simulink model "Kirov_physics"  (R2024b)
settings: Solver=FixedStepDiscrete  StartTime=0.0  StopTime=inf  FixedStep=dt  RelTol=1e-3
undefined symbols (not defined in the file): accel_O, airspeed_bp, alpha_B, alpha_bp, alphaFull, alphaOff, b, battery_capacity_bp, battery_current_bp, battery_initial_capacity_mAh, battery_voltage_table, beta_bp, betaFull, betaOff, brake, brakes, c, channels, CLa, Clb, Clp, CLq, Clr, Cma, Cmq, Cnb, Cnp, Cnr, current_table, DiscIntNeverNeededParam, dt, ELEV_bp, elevator, f, flap, flaps, FLAPS_bp, gear, heightFadeStart, heightOff, hgt_0, Inertia_body, Inertia_load, kInduced, L_aileron, L_throttle, LAILE_bp, lat_0, lon_0, M_aile, M_body, M_elev, M_flap, M_front_gear, M_load, M_main_gear, M_prop, M_rudd, M_spoiler, minWingHeight ... (+36)
libraries: sm_lib x673, simulink x58, nesl_utility x51, simulink_extras x24, uavmavlinklib x12, instrumentlib x4, vrlib x3, aerolibfltsims x3, sharedtransform x3, eeGeneralControl x2, aerolibutil x2, AP_Connector x2
(part 6 of 6)

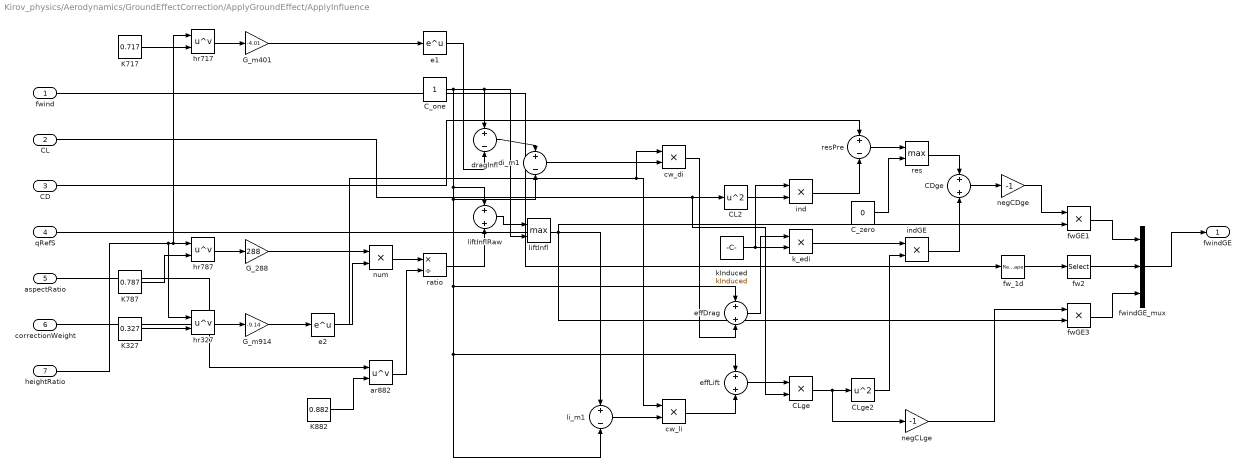
== system Kirov_physics/Aerodynamics/GroundEffectCorrection/ApplyGroundEffect/ApplyInfluence ==
  fwind : Inport
  CL : Inport  Port=2
  CD : Inport  Port=3
  qRefS : Inport  Port=4
  aspectRatio : Inport  Port=5
  correctionWeight : Inport  Port=6
  heightRatio : Inport  Port=7
  CDge : Sum
  CL2 : Math  Operator=square
  CLge : Product
  CLge2 : Math  Operator=square
  C_one : Constant
  C_zero : Constant  Value=0
  G_288 : Gain  Gain=288
  G_m401 : Gain  Gain=-4.01
  G_m914 : Gain  Gain=-9.14
  K327 : Constant  Value=0.327
  K717 : Constant  Value=0.717
  K787 : Constant  Value=0.787
  K882 : Constant  Value=0.882
  ar882 : Math  Operator=pow
  cw_di : Product
  cw_li : Product
  di_m1 : Sum  Inputs=+-
  dragInfl : Sum  Inputs=+-
  e1 : Math
  e2 : Math
  effDrag : Sum
  effLift : Sum
  fw2 : Selector  InputPortWidth=3  IndexOptions=Index vector (dialog)  Indices=[2]  OutputSizes=1
  fwGE1 : Product
  fwGE3 : Product
  fw_1d : Reshape
  fwindGE_mux : Mux  Inputs=3
  hr327 : Math  Operator=pow
  hr717 : Math  Operator=pow
  hr787 : Math  Operator=pow
  ind : Product
  indGE : Product
  kInduced : Constant  Value=kInduced
  k_edi : Product
  li_m1 : Sum  Inputs=+-
  liftInfl : MinMax  Function=max  Inputs=2
  liftInflRaw : Sum
  negCDge : Gain  Gain=-1
  negCLge : Gain  Gain=-1
  num : Product
  ratio : Product  Inputs=*/
  res : MinMax  Function=max  Inputs=2
  resPre : Sum  Inputs=+-
  fwindGE : Outport
  wires:
  hr717/1 -> G_m401/1
  fwGE3/1 -> fwindGE_mux/3
  CL2/1 -> ind/2
  heightRatio/1 -> hr327/1, hr717/1, hr787/1
  C_one/1 -> effLift/1, li_m1/2, effDrag/1, di_m1/2, liftInflRaw/1, liftInfl/2, dragInfl/1
  K717/1 -> hr717/2
  K787/1 -> hr787/2
  CLge2/1 -> indGE/2
  K327/1 -> hr327/2
  negCLge/1 -> fwGE3/1
  hr787/1 -> G_288/1
  hr327/1 -> G_m914/1
  G_m401/1 -> e1/1
  G_288/1 -> num/1
  G_m914/1 -> e2/1
  li_m1/1 -> cw_li/2
  e2/1 -> num/2
  aspectRatio/1 -> ar882/1
  K882/1 -> ar882/2
  ind/1 -> resPre/2
  num/1 -> ratio/1
  kInduced/1 -> k_edi/2, ind/1
  ar882/1 -> ratio/2
  e1/1 -> dragInfl/2
  CLge/1 -> negCLge/1, CLge2/1
  ratio/1 -> liftInflRaw/2
  dragInfl/1 -> di_m1/1
  liftInflRaw/1 -> liftInfl/1
  indGE/1 -> CDge/2
  di_m1/1 -> cw_di/2
  fwindGE_mux/1 -> fwindGE/1
  liftInfl/1 -> li_m1/1
  correctionWeight/1 -> cw_di/1, cw_li/1
  resPre/1 -> res/1
  cw_di/1 -> effDrag/2
  CL/1 -> CLge/2, CL2/1
  cw_li/1 -> effLift/2
  effDrag/1 -> k_edi/1
  effLift/1 -> CLge/1
  CD/1 -> resPre/1
  k_edi/1 -> indGE/1
  C_zero/1 -> res/2
  res/1 -> CDge/1
  CDge/1 -> negCDge/1
  fwind/1 -> fw_1d/1
  negCDge/1 -> fwGE1/1
  fw_1d/1 -> fw2/1
  qRefS/1 -> fwGE1/2, fwGE3/2
  fwGE1/1 -> fwindGE_mux/1
  fw2/1 -> fwindGE_mux/2

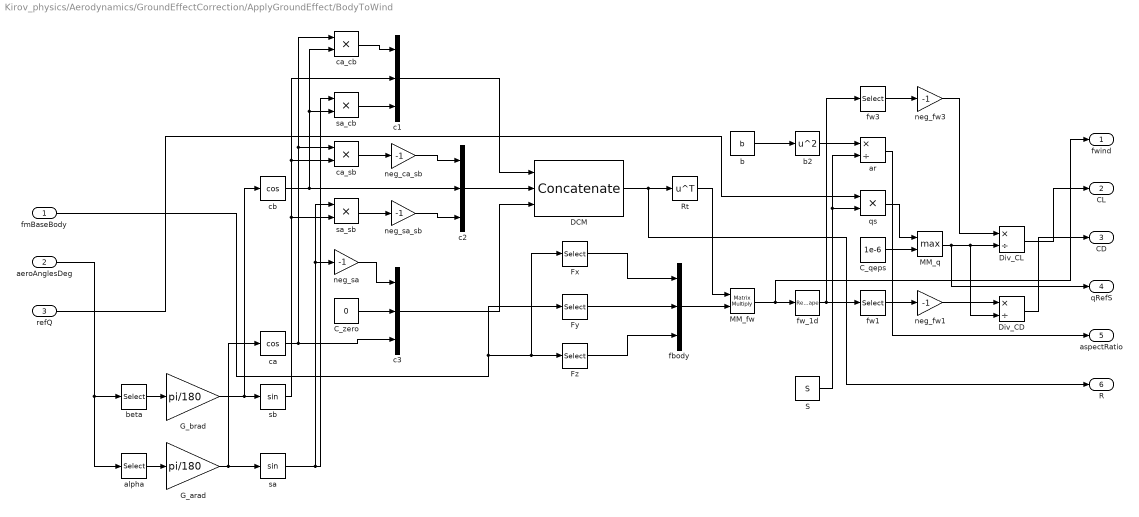
== system Kirov_physics/Aerodynamics/GroundEffectCorrection/ApplyGroundEffect/BodyToWind ==
  fmBaseBody : Inport
  aeroAnglesDeg : Inport  Port=2
  refQ : Inport  Port=3
  C_qeps : Constant  Value=1e-6
  C_zero : Constant  Value=0
  DCM : Concatenate  NumInputs=3  Mode=Multidimensional array  ConcatenateDimension=2
  Div_CD : Product  Inputs=*/
  Div_CL : Product  Inputs=*/
  Fx : Selector  InputPortWidth=6  IndexOptions=Index vector (dialog)  Indices=[1]  OutputSizes=1
  Fy : Selector  InputPortWidth=6  IndexOptions=Index vector (dialog)  Indices=[2]  OutputSizes=1
  Fz : Selector  InputPortWidth=6  IndexOptions=Index vector (dialog)  Indices=[3]  OutputSizes=1
  G_arad : Gain  Gain=pi/180
  G_brad : Gain  Gain=pi/180
  MM_fw : Product  Multiplication=Matrix(*)
  MM_q : MinMax  Function=max  Inputs=2
  Rt : Math  Operator=transpose
  S : Constant  Value=S
  alpha : Selector  InputPortWidth=2  IndexOptions=Index vector (dialog)  Indices=[1]  OutputSizes=1
  ar : Product  Inputs=*/
  b : Constant  Value=b
  b2 : Math  Operator=square
  beta : Selector  InputPortWidth=2  IndexOptions=Index vector (dialog)  Indices=[2]  OutputSizes=1
  c1 : Mux  Inputs=3
  c2 : Mux  Inputs=3
  c3 : Mux  Inputs=3
  ca : Trigonometry  Operator=cos
  ca_cb : Product
  ca_sb : Product
  cb : Trigonometry  Operator=cos
  fbody : Mux  Inputs=3
  fw1 : Selector  InputPortWidth=3  IndexOptions=Index vector (dialog)  Indices=[1]  OutputSizes=1
  fw3 : Selector  InputPortWidth=3  IndexOptions=Index vector (dialog)  Indices=[3]  OutputSizes=1
  fw_1d : Reshape
  neg_ca_sb : Gain  Gain=-1
  neg_fw1 : Gain  Gain=-1
  neg_fw3 : Gain  Gain=-1
  neg_sa : Gain  Gain=-1
  neg_sa_sb : Gain  Gain=-1
  qs : Product
  sa : Trigonometry
  sa_cb : Product
  sa_sb : Product
  sb : Trigonometry
  fwind : Outport
  CL : Outport  Port=2
  CD : Outport  Port=3
  qRefS : Outport  Port=4
  aspectRatio : Outport  Port=5
  R : Outport  Port=6
  wires:
  G_brad/1 -> cb/1, sb/1
  aeroAnglesDeg/1 -> alpha/1, beta/1
  Div_CL/1 -> CL/1
  beta/1 -> G_brad/1
  sb/1 -> c1/2, ca_sb/2, sa_sb/2
  alpha/1 -> G_arad/1
  cb/1 -> ca_cb/2, sa_cb/2, c2/2
  G_arad/1 -> sa/1, ca/1
  ca/1 -> ca_sb/1, ca_cb/1, c3/3
  b/1 -> b2/1
  sa/1 -> sa_sb/1, neg_sa/1, sa_cb/1
  ca_cb/1 -> c1/1
  sa_cb/1 -> c1/3
  C_zero/1 -> c3/2
  ca_sb/1 -> neg_ca_sb/1
  Fx/1 -> fbody/1
  sa_sb/1 -> neg_sa_sb/1
  neg_sa/1 -> c3/1
  c1/1 -> DCM/1
  neg_ca_sb/1 -> c2/1
  neg_sa_sb/1 -> c2/3
  C_qeps/1 -> MM_q/2
  c3/1 -> DCM/3
  c2/1 -> DCM/2
  fmBaseBody/1 -> Fx/1, Fz/1, Fy/1
  DCM/1 -> Rt/1, R/1
  MM_q/1 -> Div_CD/2, Div_CL/2, qRefS/1
  Fy/1 -> fbody/2
  Fz/1 -> fbody/3
  Rt/1 -> MM_fw/1
  fbody/1 -> MM_fw/2
  MM_fw/1 -> fw_1d/1, fwind/1
  Div_CD/1 -> CD/1
  b2/1 -> ar/1
  fw_1d/1 -> fw1/1, fw3/1
  S/1 -> ar/2, qs/2
  refQ/1 -> qs/1
  fw3/1 -> neg_fw3/1
  ar/1 -> aspectRatio/1
  qs/1 -> MM_q/1
  fw1/1 -> neg_fw1/1
  neg_fw3/1 -> Div_CL/1
  neg_fw1/1 -> Div_CD/1

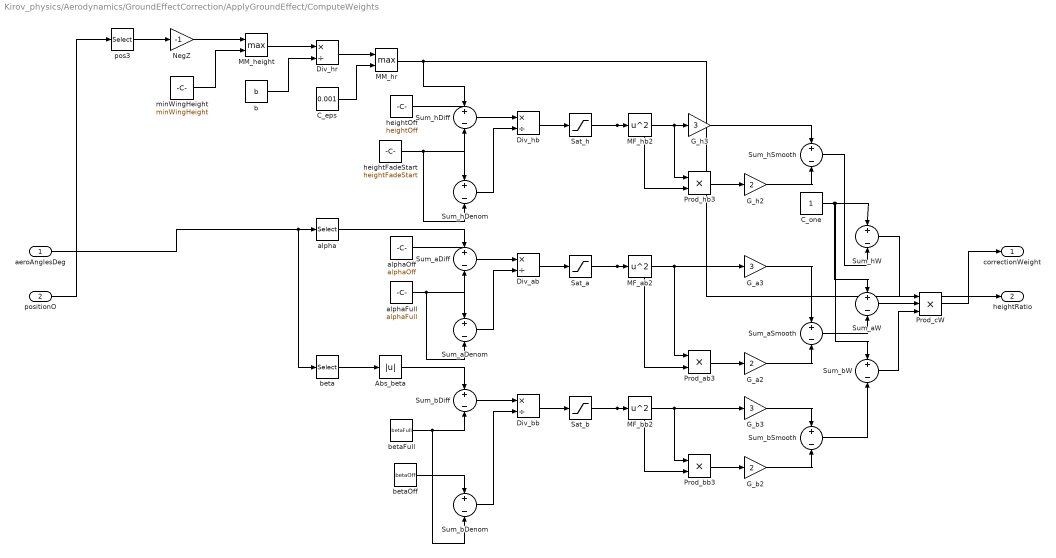
== system Kirov_physics/Aerodynamics/GroundEffectCorrection/ApplyGroundEffect/ComputeWeights ==
  aeroAnglesDeg : Inport
  positionO : Inport  Port=2
  Abs_beta : Abs  SaturateOnIntegerOverflow=off
  C_eps : Constant  Value=0.001
  C_one : Constant
  Div_ab : Product  Inputs=*/
  Div_bb : Product  Inputs=*/
  Div_hb : Product  Inputs=*/
  Div_hr : Product  Inputs=*/
  G_a2 : Gain  Gain=2
  G_a3 : Gain  Gain=3
  G_b2 : Gain  Gain=2
  G_b3 : Gain  Gain=3
  G_h2 : Gain  Gain=2
  G_h3 : Gain  Gain=3
  MF_ab2 : Math  Operator=square
  MF_bb2 : Math  Operator=square
  MF_hb2 : Math  Operator=square
  MM_height : MinMax  Function=max  Inputs=2
  MM_hr : MinMax  Function=max  Inputs=2
  NegZ : Gain  Gain=-1
  Prod_ab3 : Product
  Prod_bb3 : Product
  Prod_cW : Product  Inputs=3
  Prod_hb3 : Product
  Sat_a : Saturate  UpperLimit=1  LowerLimit=0
  Sat_b : Saturate  UpperLimit=1  LowerLimit=0
  Sat_h : Saturate  UpperLimit=1  LowerLimit=0
  Sum_aDenom : Sum  Inputs=+-
  Sum_aDiff : Sum  Inputs=+-
  Sum_aSmooth : Sum  Inputs=+-
  Sum_aW : Sum  Inputs=+-
  Sum_bDenom : Sum  Inputs=+-
  Sum_bDiff : Sum  Inputs=+-
  Sum_bSmooth : Sum  Inputs=+-
  Sum_bW : Sum  Inputs=+-
  Sum_hDenom : Sum  Inputs=+-
  Sum_hDiff : Sum  Inputs=+-
  Sum_hSmooth : Sum  Inputs=+-
  Sum_hW : Sum  Inputs=+-
  alpha : Selector  InputPortWidth=2  IndexOptions=Index vector (dialog)  Indices=[1]  OutputSizes=1
  alphaFull : Constant  Value=alphaFull
  alphaOff : Constant  Value=alphaOff
  b : Constant  Value=b
  beta : Selector  InputPortWidth=2  IndexOptions=Index vector (dialog)  Indices=[2]  OutputSizes=1
  betaFull : Constant  Value=betaFull
  betaOff : Constant  Value=betaOff
  heightFadeStart : Constant  Value=heightFadeStart
  heightOff : Constant  Value=heightOff
  minWingHeight : Constant  Value=minWingHeight
  pos3 : Selector  InputPortWidth=3  IndexOptions=Index vector (dialog)  Indices=[3]  OutputSizes=1
  correctionWeight : Outport
  heightRatio : Outport  Port=2
  wires:
  b/1 -> Div_hr/2
  G_b2/1 -> Sum_bSmooth/2
  Prod_ab3/1 -> G_a2/1
  pos3/1 -> NegZ/1
  positionO/1 -> pos3/1
  G_a3/1 -> Sum_aSmooth/1
  NegZ/1 -> MM_height/1
  minWingHeight/1 -> MM_height/2
  MM_height/1 -> Div_hr/1
  Sum_hDiff/1 -> Div_hb/1
  aeroAnglesDeg/1 -> alpha/1, beta/1
  betaOff/1 -> Sum_bDenom/1
  Div_hr/1 -> MM_hr/1
  C_eps/1 -> MM_hr/2
  Div_ab/1 -> Sat_a/1
  alpha/1 -> Sum_aDiff/1
  Div_hb/1 -> Sat_h/1
  beta/1 -> Abs_beta/1
  MM_hr/1 -> Sum_hDiff/1, heightRatio/1
  G_a2/1 -> Sum_aSmooth/2
  MF_hb2/1 -> G_h3/1, Prod_hb3/1
  Sum_bDenom/1 -> Div_bb/2
  heightOff/1 -> Sum_hDenom/1
  heightFadeStart/1 -> Sum_hDenom/2, Sum_hDiff/2
  Div_bb/1 -> Sat_b/1
  alphaOff/1 -> Sum_aDenom/1
  alphaFull/1 -> Sum_aDiff/2, Sum_aDenom/2
  Sum_hSmooth/1 -> Sum_hW/2
  Abs_beta/1 -> Sum_bDiff/1
  betaFull/1 -> Sum_bDenom/2, Sum_bDiff/2
  Sum_hDenom/1 -> Div_hb/2
  Prod_hb3/1 -> G_h2/1
  Sum_aDiff/1 -> Div_ab/1
  Sum_aDenom/1 -> Div_ab/2
  Sum_bDiff/1 -> Div_bb/1
  Sum_hW/1 -> Prod_cW/1
  C_one/1 -> Sum_hW/1, Sum_bW/1, Sum_aW/1
  Sat_h/1 -> Prod_hb3/2, MF_hb2/1
  Sat_a/1 -> Prod_ab3/2, MF_ab2/1
  Sat_b/1 -> MF_bb2/1, Prod_bb3/2
  MF_ab2/1 -> G_a3/1, Prod_ab3/1
  MF_bb2/1 -> Prod_bb3/1, G_b3/1
  Prod_cW/1 -> correctionWeight/1
  G_h3/1 -> Sum_hSmooth/1
  Prod_bb3/1 -> G_b2/1
  G_h2/1 -> Sum_hSmooth/2
  Sum_bSmooth/1 -> Sum_bW/2
  G_b3/1 -> Sum_bSmooth/1
  Sum_aSmooth/1 -> Sum_aW/2
  Sum_aW/1 -> Prod_cW/2
  Sum_bW/1 -> Prod_cW/3

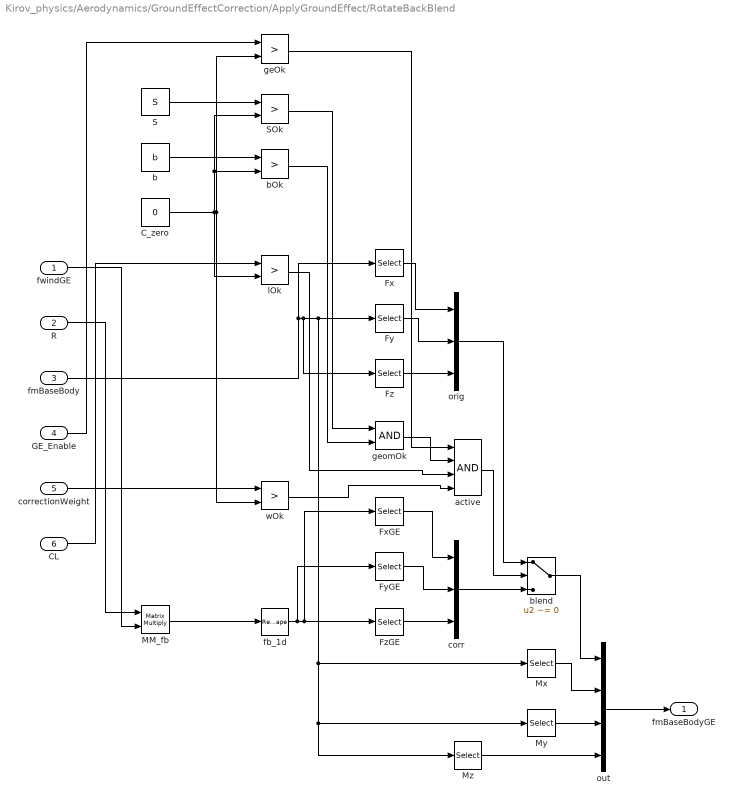
== system Kirov_physics/Aerodynamics/GroundEffectCorrection/ApplyGroundEffect/RotateBackBlend ==
  fwindGE : Inport
  R : Inport  Port=2
  fmBaseBody : Inport  Port=3
  GE_Enable : Inport  Port=4
  correctionWeight : Inport  Port=5
  CL : Inport  Port=6
  C_zero : Constant  Value=0
  Fx : Selector  InputPortWidth=6  IndexOptions=Index vector (dialog)  Indices=[1]  OutputSizes=1
  FxGE : Selector  InputPortWidth=3  IndexOptions=Index vector (dialog)  Indices=[1]  OutputSizes=1
  Fy : Selector  InputPortWidth=6  IndexOptions=Index vector (dialog)  Indices=[2]  OutputSizes=1
  FyGE : Selector  InputPortWidth=3  IndexOptions=Index vector (dialog)  Indices=[2]  OutputSizes=1
  Fz : Selector  InputPortWidth=6  IndexOptions=Index vector (dialog)  Indices=[3]  OutputSizes=1
  FzGE : Selector  InputPortWidth=3  IndexOptions=Index vector (dialog)  Indices=[3]  OutputSizes=1
  MM_fb : Product  Multiplication=Matrix(*)
  Mx : Selector  InputPortWidth=6  IndexOptions=Index vector (dialog)  Indices=[4]  OutputSizes=1
  My : Selector  InputPortWidth=6  IndexOptions=Index vector (dialog)  Indices=[5]  OutputSizes=1
  Mz : Selector  InputPortWidth=6  IndexOptions=Index vector (dialog)  Indices=[6]  OutputSizes=1
  S : Constant  Value=S
  SOk : RelationalOperator  Operator=>  OutDataTypeStr=boolean  RndMeth=Simplest  InputSameDT=off
  active : Logic  Inputs=4  AllPortsSameDT=off  OutDataTypeStr=boolean
  b : Constant  Value=b
  bOk : RelationalOperator  Operator=>  OutDataTypeStr=boolean  RndMeth=Simplest  InputSameDT=off
  blend : Switch  Criteria=u2 ~= 0  Threshold=0.5  SaturateOnIntegerOverflow=off  InputSameDT=off
  corr : Mux  Inputs=3
  fb_1d : Reshape
  geOk : RelationalOperator  Operator=>  OutDataTypeStr=boolean  RndMeth=Simplest  InputSameDT=off
  geomOk : Logic  AllPortsSameDT=off  OutDataTypeStr=boolean
  lOk : RelationalOperator  Operator=>  OutDataTypeStr=boolean  RndMeth=Simplest  InputSameDT=off
  orig : Mux  Inputs=3
  out : Mux
  wOk : RelationalOperator  Operator=>  OutDataTypeStr=boolean  RndMeth=Simplest  InputSameDT=off
  fmBaseBodyGE : Outport
  wires:
  R/1 -> MM_fb/1
  Fx/1 -> orig/1
  b/1 -> bOk/1
  fwindGE/1 -> MM_fb/2
  GE_Enable/1 -> geOk/1
  S/1 -> SOk/1
  C_zero/1 -> geOk/2, wOk/2, SOk/2, bOk/2, lOk/2
  CL/1 -> lOk/1
  correctionWeight/1 -> wOk/1
  MM_fb/1 -> fb_1d/1
  geOk/1 -> active/1
  SOk/1 -> geomOk/1
  wOk/1 -> active/4
  bOk/1 -> geomOk/2
  lOk/1 -> active/3
  orig/1 -> blend/1
  fmBaseBody/1 -> Fx/1, Mz/1, My/1, Mx/1, Fy/1, Fz/1
  fb_1d/1 -> FzGE/1, FxGE/1, FyGE/1
  Fy/1 -> orig/2
  Fz/1 -> orig/3
  geomOk/1 -> active/2
  FxGE/1 -> corr/1
  FyGE/1 -> corr/2
  FzGE/1 -> corr/3
  active/1 -> blend/2
  corr/1 -> blend/3
  Mz/1 -> out/4
  blend/1 -> out/1
  Mx/1 -> out/2
  My/1 -> out/3
  out/1 -> fmBaseBodyGE/1

== system Kirov_physics/SendState/Mavlink/Mission_Server/Send_Mission_Count ==
  Enable : EnablePort
  Mission_Count_Blank : uavmavlinklib/MAVLink Blank Message  dialectSource=Select from standard MAVLink dialects  dialect=common.xml  dialectCustom=common.xml  version=2  messageType=MISSION_COUNT  SystemID=1  ComponentID=1  SampleTime=-1
  Mission_Count_Serializer : uavmavlinklib/MAVLink Serializer  dialectSource=Select from standard MAVLink dialects  dialect=common.xml  dialectCustom=common.xml  version=2  messageType=MISSION_COUNT
  Mission_Item_Count : Constant  Value=uint16(4)  OutDataTypeStr=uint16
  Mission_Type : Constant  Value=uint8(0)  OutDataTypeStr=uint8
  QGC_Component_ID : Constant  Value=uint8(190)  OutDataTypeStr=uint8
  QGC_System_ID : Constant  Value=uint8(255)  OutDataTypeStr=uint8
  Set_Mission_Count : BusAssignment  AssignedSignals=Payload.target_system,Payload.target_component,Payload.count,Payload.mission_type
  UDP_Send_Mission_Count : instrumentlib/UDP Send  Host=127.0.0.1  Port=14550  LocalAddress=0.0.0.0  LocalPort=14560  EnablePortSharing=on  OutputDatagramPacketSize=280  ByteOrder=big-endian  EnableBlockingMode=off  SimulateUsing=Interpreted execution
  Unused_Frame_Length : Terminator
  wires:
  Mission_Count_Blank/1 -> Set_Mission_Count/1
  QGC_Component_ID/1 -> Set_Mission_Count/3
  QGC_System_ID/1 -> Set_Mission_Count/2
  Mission_Type/1 -> Set_Mission_Count/5
  Mission_Item_Count/1 -> Set_Mission_Count/4
  Set_Mission_Count/1 -> Mission_Count_Serializer/1
  Mission_Count_Serializer/2 -> Unused_Frame_Length/1
  Mission_Count_Serializer/1 -> UDP_Send_Mission_Count/1

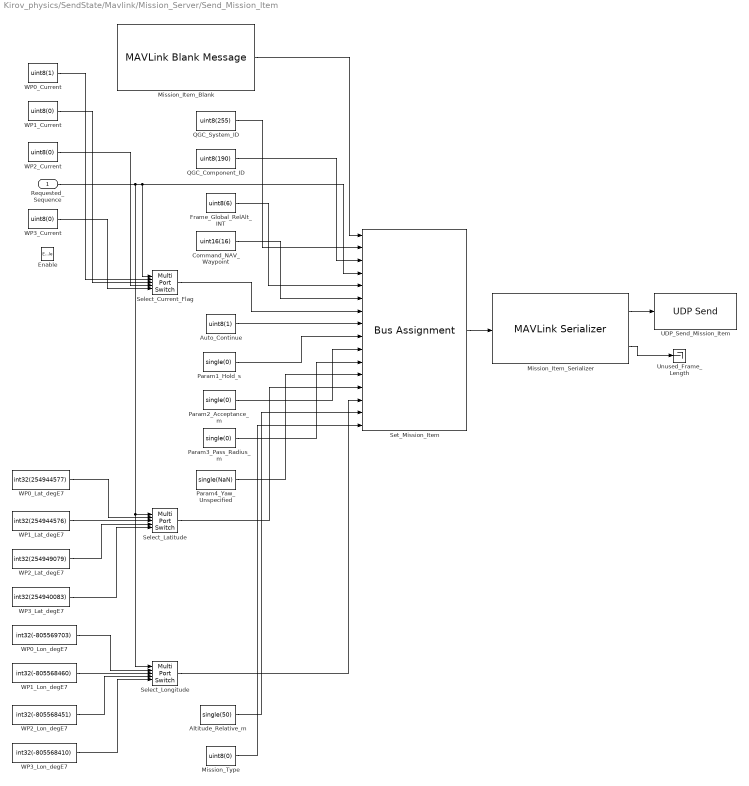
== system Kirov_physics/SendState/Mavlink/Mission_Server/Send_Mission_Item ==
  Requested_Sequence : Inport
  Enable : EnablePort
  Altitude_Relative_m : Constant  Value=single(50)  OutDataTypeStr=single
  Auto_Continue : Constant  Value=uint8(1)  OutDataTypeStr=uint8
  Command_NAV_Waypoint : Constant  Value=uint16(16)  OutDataTypeStr=uint16
  Frame_Global_RelAlt_INT : Constant  Value=uint8(6)  OutDataTypeStr=uint8
  Mission_Item_Blank : uavmavlinklib/MAVLink Blank Message  dialectSource=Select from standard MAVLink dialects  dialect=common.xml  dialectCustom=common.xml  version=2  messageType=MISSION_ITEM_INT  SystemID=1  ComponentID=1  SampleTime=-1
  Mission_Item_Serializer : uavmavlinklib/MAVLink Serializer  dialectSource=Select from standard MAVLink dialects  dialect=common.xml  dialectCustom=common.xml  version=2  messageType=MISSION_ITEM_INT
  Mission_Type : Constant  Value=uint8(0)  OutDataTypeStr=uint8
  Param1_Hold_s : Constant  Value=single(0)  OutDataTypeStr=single
  Param2_Acceptance_m : Constant  Value=single(0)  OutDataTypeStr=single
  Param3_Pass_Radius_m : Constant  Value=single(0)  OutDataTypeStr=single
  Param4_Yaw_Unspecified : Constant  Value=single(NaN)  OutDataTypeStr=single
  QGC_Component_ID : Constant  Value=uint8(190)  OutDataTypeStr=uint8
  QGC_System_ID : Constant  Value=uint8(255)  OutDataTypeStr=uint8
  Select_Current_Flag : MultiPortSwitch  DataPortOrder=Zero-based contiguous  Inputs=4  zeroidx=on  OutDataTypeStr=uint8  SaturateOnIntegerOverflow=off  InputSameDT=off
  Select_Latitude : MultiPortSwitch  DataPortOrder=Zero-based contiguous  Inputs=4  zeroidx=on  OutDataTypeStr=int32  SaturateOnIntegerOverflow=off  InputSameDT=off
  Select_Longitude : MultiPortSwitch  DataPortOrder=Zero-based contiguous  Inputs=4  zeroidx=on  OutDataTypeStr=int32  SaturateOnIntegerOverflow=off  InputSameDT=off
  Set_Mission_Item : BusAssignment  AssignedSignals=Payload.target_system,Payload.target_component,Payload.seq,Payload.frame,Payload.command,Payload.current,Payload.autocontinue,Payload.param1,Payload.param2,Payload.param3,Payload.param4,Payload.x,Payload.y,Payload.z,Payload.mission_type
  UDP_Send_Mission_Item : instrumentlib/UDP Send  Host=127.0.0.1  Port=14550  LocalAddress=0.0.0.0  LocalPort=14560  EnablePortSharing=on  OutputDatagramPacketSize=280  ByteOrder=big-endian  EnableBlockingMode=off  SimulateUsing=Interpreted execution
  Unused_Frame_Length : Terminator
  WP0_Current : Constant  Value=uint8(1)  OutDataTypeStr=uint8
  WP0_Lat_degE7 : Constant  Value=int32(254944577)  OutDataTypeStr=int32
  WP0_Lon_degE7 : Constant  Value=int32(-805569703)  OutDataTypeStr=int32
  WP1_Current : Constant  Value=uint8(0)  OutDataTypeStr=uint8
  WP1_Lat_degE7 : Constant  Value=int32(254944576)  OutDataTypeStr=int32
  WP1_Lon_degE7 : Constant  Value=int32(-805568460)  OutDataTypeStr=int32
  WP2_Current : Constant  Value=uint8(0)  OutDataTypeStr=uint8
  WP2_Lat_degE7 : Constant  Value=int32(254949079)  OutDataTypeStr=int32
  WP2_Lon_degE7 : Constant  Value=int32(-805568451)  OutDataTypeStr=int32
  WP3_Current : Constant  Value=uint8(0)  OutDataTypeStr=uint8
  WP3_Lat_degE7 : Constant  Value=int32(254940083)  OutDataTypeStr=int32
  WP3_Lon_degE7 : Constant  Value=int32(-805568410)  OutDataTypeStr=int32
  wires:
  WP0_Current/1 -> Select_Current_Flag/2
  WP1_Current/1 -> Select_Current_Flag/3
  WP2_Current/1 -> Select_Current_Flag/4
  WP3_Current/1 -> Select_Current_Flag/5
  Requested_Sequence/1 -> Select_Longitude/1, Select_Latitude/1, Set_Mission_Item/4, Select_Current_Flag/1
  WP0_Lat_degE7/1 -> Select_Latitude/2
  WP1_Lat_degE7/1 -> Select_Latitude/3
  WP3_Lat_degE7/1 -> Select_Latitude/5
  WP2_Lat_degE7/1 -> Select_Latitude/4
  WP1_Lon_degE7/1 -> Select_Longitude/3
  WP0_Lon_degE7/1 -> Select_Longitude/2
  WP3_Lon_degE7/1 -> Select_Longitude/5
  WP2_Lon_degE7/1 -> Select_Longitude/4
  Mission_Item_Blank/1 -> Set_Mission_Item/1
  QGC_System_ID/1 -> Set_Mission_Item/2
  Frame_Global_RelAlt_INT/1 -> Set_Mission_Item/5
  QGC_Component_ID/1 -> Set_Mission_Item/3
  Auto_Continue/1 -> Set_Mission_Item/8
  Command_NAV_Waypoint/1 -> Set_Mission_Item/6
  Select_Current_Flag/1 -> Set_Mission_Item/7
  Param2_Acceptance_m/1 -> Set_Mission_Item/10
  Param1_Hold_s/1 -> Set_Mission_Item/9
  Param4_Yaw_Unspecified/1 -> Set_Mission_Item/12
  Param3_Pass_Radius_m/1 -> Set_Mission_Item/11
  Select_Latitude/1 -> Set_Mission_Item/13
  Select_Longitude/1 -> Set_Mission_Item/14
  Mission_Type/1 -> Set_Mission_Item/16
  Altitude_Relative_m/1 -> Set_Mission_Item/15
  Set_Mission_Item/1 -> Mission_Item_Serializer/1
  Mission_Item_Serializer/2 -> Unused_Frame_Length/1
  Mission_Item_Serializer/1 -> UDP_Send_Mission_Item/1

== system Kirov_physics/SendState/Mavlink/WGS84/WGS84_Derivative ==
  lat_0 : Inport
  h_0 : Inport  Port=2
  Add : Sum
  Add1 : Sum
  Divide : Product  Inputs=*/
  Product{,1..4} (5 alike) : Product  RndMeth=Zero
  Subtract : Sum  Inputs=+-
  Subtract1 : Sum  Inputs=-+
  Subtract2 : Sum  Inputs=+-
  Trigonometric Function : Trigonometry
  Trigonometric Function1 : Trigonometry  Operator=cos
  Trigonometric Function2 : Trigonometry  Operator=cos
  b : Constant  Value=1/298.257
  c : Constant
  constant : Constant  Value=2
  constant1 : Constant  Value=-1
  constant2 : Constant
  earth_radius : Constant  Value=6378137
  sqrt : Math  Operator=sqrt  SignedPower=on
  u^1 : Math  Operator=square  SignedPower=on
  u^2 : Math  Operator=square  SignedPower=on
  dx_dlat : Outport  VectorParamsAs1DForOutWhenUnconnected=off
  dy_dlon : Outport  Port=2  VectorParamsAs1DForOutWhenUnconnected=off
  dz_dh : Outport  Port=3  InitialOutput=1  VectorParamsAs1DForOutWhenUnconnected=off
  wires:
  constant1/1 -> dz_dh/1
  Product4/1 -> dy_dlon/1
  Add1/1 -> Product4/1
  Trigonometric Function2/1 -> Product4/2
  Product3/1 -> Add/1
  Subtract2/1 -> Product3/1
  Product2/1 -> Subtract2/2
  u^1/1 -> Product2/1
  Trigonometric Function1/1 -> u^1/1
  constant2/1 -> Subtract2/1
  h_0/1 -> Add1/1, Add/2
  Add/1 -> dx_dlat/1
  Divide/1 -> Product3/2, Add1/2
  sqrt/1 -> Divide/2
  Product1/1 -> Product2/2, Product/1
  Subtract1/1 -> Product1/2
  constant/1 -> Subtract1/2
  b/1 -> Subtract1/1, Product1/1
  Product/1 -> Subtract/2
  Subtract/1 -> sqrt/1
  c/1 -> Subtract/1
  u^2/1 -> Product/2
  Trigonometric Function/1 -> u^2/1
  lat_0/1 -> Trigonometric Function2/1, Trigonometric Function/1, Trigonometric Function1/1
  earth_radius/1 -> Divide/1

== system Kirov_physics/SendState/Mavlink/WGS84/Zero_Value_Exclusion ==
  u : Inport
  Abs : Abs  SaturateOnIntegerOverflow=off
  Constant : Constant
  Product : Product  RndMeth=Zero
  Saturation : Saturate  UpperLimit=10e7  LowerLimit=1e-6  LinearizeAsGain=off
  Sign : Signum
  Switch : Switch  Criteria=u2 ~= 0  SaturateOnIntegerOverflow=off  InputSameDT=off
  y : Outport  VectorParamsAs1DForOutWhenUnconnected=off
  wires:
  u/1 -> Sign/1, Abs/1
  Abs/1 -> Saturation/1
  Saturation/1 -> Product/1
  Sign/1 -> Switch/2, Switch/1
  Product/1 -> y/1
  Switch/1 -> Product/2
  Constant/1 -> Switch/3

== matlab function Kirov_physics/Referee/MATLAB Function1 ==
  data: u input; y output
function y = fcn(u)
if u == true
    disp('Fly over safety zone!')
end
y = u;

== matlab function Kirov_physics/Aerodynamics/Wind2Body/MATLAB Function ==
  data: fmWind input; fmBody output; aeroAnglesDeg input
function fmBody = windToBodyFM(fmWind, aeroAnglesDeg)
%#codegen
% fmWind         = [Fx Fy Fz Mx My Mz]，风轴系
% aeroAnglesDeg  = [alpha beta]，单位 deg
% fmBody         = [Fx Fy Fz Mx My Mz]，体轴系
%
% 坐标约定：
% x 向前，y 向右，z 向下

alpha = aeroAnglesDeg(1) * pi / 180;
beta  = aeroAnglesDeg(2) * pi / 180;

ca = cos(alpha);
sa = sin(alpha);
cb = cos(beta);
sb = sin(beta);

FxW = fmWind(1);
FyW = fmWind(2);
FzW = fmWind(3);

MxW = fmWind(4);
MyW = fmWind(5);
MzW = fmWind(6);

% 风轴系力转换到体轴系
FxB = ca*cb*FxW - ca*sb*FyW - sa*FzW;
FyB =    sb*FxW +    cb*FyW;
FzB = sa*cb*FxW - sa*sb*FyW + ca*FzW;

% 风轴系力矩转换到体轴系
MxB = ca*cb*MxW - ca*sb*MyW - sa*MzW;
MyB =    sb*MxW +    cb*MyW;
MzB = sa*cb*MxW - sa*sb*MyW + ca*MzW;

fmBody = [FxB, FyB, FzB, MxB, MyB, MzB];

end

== matlab function Kirov_physics/Dynamics/MATLAB Function ==
  data: targetNED input; q output; cameraNED input
function q = cameraPointingAngle(targetNED, cameraNED)

d = targetNED - cameraNED;

dN = d(1);
dE = d(2);
dD = d(3);

yaw   = atan2(dE, dN);
pitch = atan2(-dD, hypot(dN, dE));
roll  = 0;

% Gimbal Joint输入：qx、qy、qz
q = [roll; pitch; yaw];

end
